simulink model "assignment4"  (R2026a)
settings: Solver=VariableStepAuto  StopTime=25  MaxStep=0.01
values from neighbouring files (symbols this model uses):
  a = 1    [assignment4_param.m]
  a_m = 1    [assignment4_param.m]
settings Model: Creator=saradenti  LastModifiedBy=saradenti

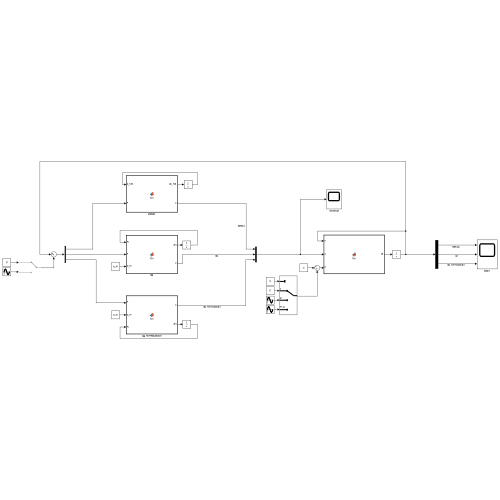
[thumbnail: Simulink's stored preview of the top-level diagram]
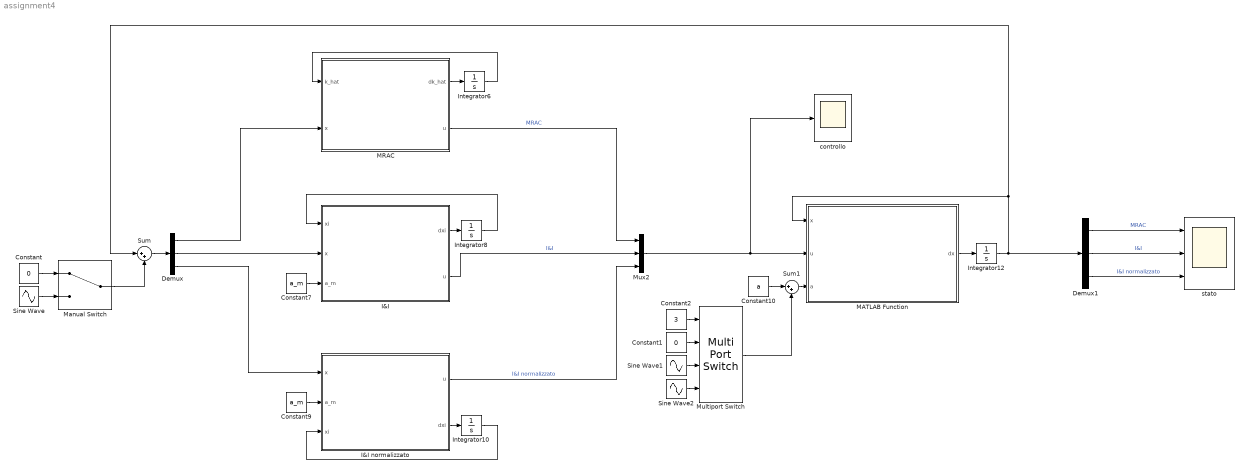
== system assignment4 ==
  Constant : Constant  Value=0
  Constant1 : Constant  Value=0
  Constant10 : Constant  Value=a
  Constant2 : Constant  Value=3
  Constant7 : Constant  Value=a_m
  Constant9 : Constant  Value=a_m
  Demux : Demux  Outputs=3
  Demux1 : Demux  Outputs=3
  I&I : MATLAB Function  TreatAsAtomicUnit=on
  I&I normalizzato : MATLAB Function  TreatAsAtomicUnit=on
  Integrator10 : Integrator
  Integrator12 : Integrator  InitialCondition=[1; 1; 1]
  Integrator6 : Integrator
  Integrator8 : Integrator
  MATLAB Function : MATLAB Function  TreatAsAtomicUnit=on
  MRAC : MATLAB Function  TreatAsAtomicUnit=on
  Manual Switch : ManualSwitch
  Multiport Switch : MultiPortSwitch  SaturateOnIntegerOverflow=off  InputSameDT=off
  Mux2 : Mux  Inputs=3
  Sine Wave : Sin  Amplitude=0.1  Frequency=1/5  SampleTime=0
  Sine Wave1 : Sin  Amplitude=1/10  Frequency=10  SampleTime=0
  Sine Wave2 : Sin  Amplitude=10  Frequency=1/10  SampleTime=0
  Sum : Sum  Inputs=|++
  Sum1 : Sum  Inputs=|++
  controllo : Scope
      settings: ActiveDisplayYMinimum=-76.503435359565628  ActiveDisplayYMaximum=6.3562928165231307
  stato : Scope  NumInputPorts=3
      settings: ActiveDisplayYMinimum=2.4661593522711875  ActiveDisplayYMaximum=3.6840063606763191  DataLoggingVariableName=ScopeData2
  wires:
  I&I/1(dxi) -> Integrator8/1
  Integrator8/1 -> I&I/1(xi)
  I&I normalizzato/1(u) -> Mux2/3  "I&I normalizzato"
  Integrator10/1 -> I&I normalizzato/3(xi)
  I&I normalizzato/2(dxi) -> Integrator10/1
  Constant9/1 -> I&I normalizzato/2(a_m)
  Constant7/1 -> I&I/3(a_m)
  MATLAB Function/1(dx) -> Integrator12/1
  Integrator12/1 -> MATLAB Function/1(x), Sum/1, Demux1/1
  MRAC/1(dk_hat) -> Integrator6/1
  Integrator6/1 -> MRAC/1(k_hat)
  Mux2/1 -> controllo/1, MATLAB Function/2(u)
  MRAC/2(u) -> Mux2/1  "MRAC"
  I&I/2(u) -> Mux2/2  "I&I"
  Demux/1 -> MRAC/2(x)
  Demux/3 -> I&I normalizzato/1(x)
  Demux/2 -> I&I/2(x)
  Demux1/1 -> stato/1  "MRAC"
  Demux1/2 -> stato/2  "I&I"
  Demux1/3 -> stato/3  "I&I normalizzato"
  Sum/1 -> Demux/1
  Manual Switch/1 -> Sum/2
  Constant/1 -> Manual Switch/1
  Sine Wave/1 -> Manual Switch/2
  Sum1/1 -> MATLAB Function/3(a)
  Constant10/1 -> Sum1/1
  Multiport Switch/1 -> Sum1/2
  Constant1/1 -> Multiport Switch/2
  Sine Wave1/1 -> Multiport Switch/3
  Constant2/1 -> Multiport Switch/1
  Sine Wave2/1 -> Multiport Switch/4

== matlab function assignment4/I&I ==
  data: xi input; x input; a_m input; dxi output; u output
function [dxi, u] = fcn(xi, x, a_m)

    a_hat = 1/2 * x^2 + xi;
    dxi = a_m * x^2;

    u = -(a_m + a_hat) * x;

== matlab function assignment4/I&I normalizzato ==
  data: x input; a_m input; u output; xi input; dxi output
function [u, dxi] = fcn(x, a_m, xi)

    a_hat = 1/2 * log(1 + x^2) + xi;
    dxi = a_m * x^2/(1+x^2);

    u = -(a_m + a_hat) * x;

== matlab function assignment4/MRAC ==
  data: dk_hat output; k_hat input; x input; u output
function [dk_hat, u]  = fcn(k_hat, x)

    dk_hat = x(1)^2;

    u = - k_hat * x(1);

== matlab function assignment4/MATLAB Function ==
  data: x input; u input; a input; dx output
function dx = fcn(x,u, a)

    dx = zeros(3,1); %dx(1) = MRAC; dx(2) = I&I; dx(3) = I&I normalizzato

    dx = a * x + u;
